simulink model "untitled1"  (R2023b)
settings: Solver=VariableStepAuto  StartTime=0.0  StopTime=10.0  RelTol=1e-3
settings Model: Creator=hp  LastModifiedBy=hp

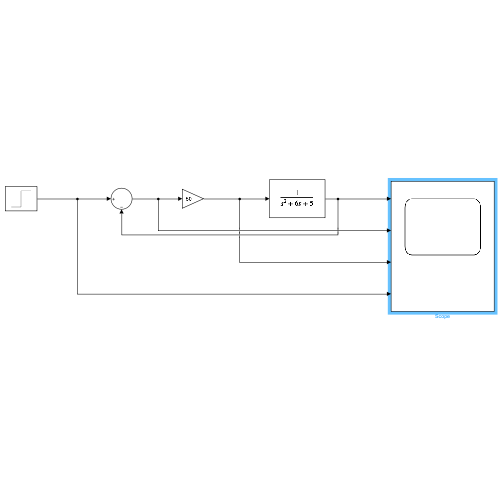
[thumbnail: Simulink's stored preview of the top-level diagram]
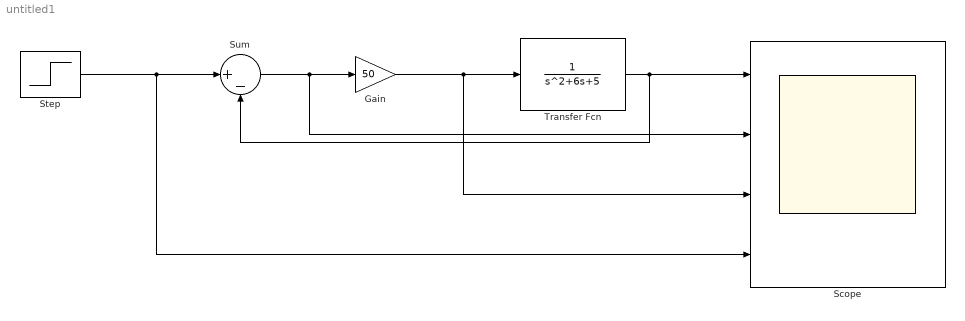
== system untitled1 ==
  Gain : Gain  Gain=50
  Scope : Scope  NumInputPorts=4
  Step : Step  SampleTime=0
  Sum : Sum  Inputs=|+-
  Transfer Fcn : TransferFcn  Denominator=[1 6 5]
  wires:
  Transfer Fcn/1 -> Scope/1, Sum/2
  Step/1 -> Scope/4, Sum/1
  Sum/1 -> Scope/2, Gain/1
  Gain/1 -> Scope/3, Transfer Fcn/1
